simulink model "J2_PMSM_SimscapeRef"  (R2026b)
settings: Solver=ode23t  StopTime=0.3  MaxStep=1e-5  RelTol=1e-6  AbsTol=1e-8
model workspace (MAT data in the model file):
  p.pp = 8
  p.Rs = 0.04675
  p.Ld = 6.15e-05
  p.Lq = 6.15e-05
  p.Kt = 0.0436218747098
  p.psi = 0.00363515622582
  p.Jm = 1.7e-05
  p.IN = 10.4269458616
  p.nmax_rpm = 6000
  p.Vdc = 24
  p.Vmax = 12.4707658145
  p.Imax = 20.9
  p.Kp = 0.386415896392
  p.Ki = 293.738913111
  p.Kaw = 760.162601626
  p.N = 100
  p.JWG = 7.9e-06
  p.s = -1
  p.Kg = 14000
  p.zeta_g = 0.05
  p.cg = 5.90423576765
  p.J_test = 7.49e-05
libraries: fl_lib x9, nesl_utility x9, sl_discontinuities x1, ee_lib x1
settings Model: Creator=rninh  LastModifiedBy=rninh
settings SimscapeCC: SimscapeLogType=all  SimscapeNominalValues="[{\"value\":\"1\",\"unit\":\"A\"},{\"value\":\"1\",\"unit\":\"bar\"},{\"value\":\"1\",\"unit\":\"cm^2\"},{\"value\":\"1\",\"unit\":\"cm^3/s\"},{\"value\":\"1\",\"unit\":\"kJ/kg\"},{\"value\":\"1\",\"unit\":\"kW\"},{\"value\":\"1\",\"unit\":\"l\"},{\"value\":\"1\",\"unit\":\"N\"},{\"value\":\"1\",\"unit\":\"N*m\"},{\"value\":\"1\",\"unit\":\"V\"},{\"value\":\"0.001\",\"unit\":\"Wb\"}]"  SimscapeUseEnergyAccounting=off

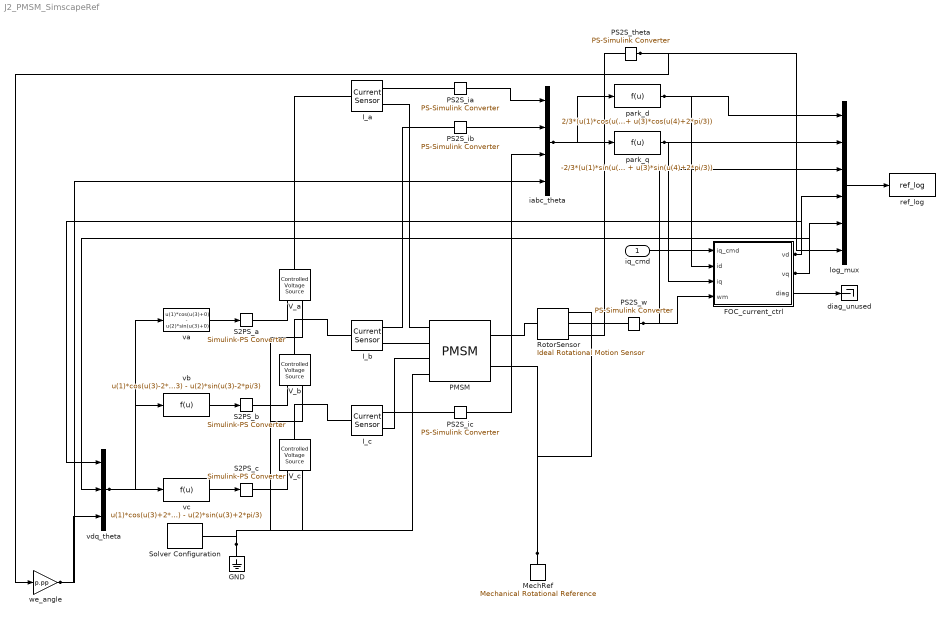
== system J2_PMSM_SimscapeRef ==
  iq_cmd : Inport  Interpolate=off
  FOC_current_ctrl : Subsystem
  GND : fl_lib/Electrical/Electrical Elements/Electrical Reference
  I_a : fl_lib/Electrical/Electrical Sensors/Current Sensor
  I_b : fl_lib/Electrical/Electrical Sensors/Current Sensor
  I_c : fl_lib/Electrical/Electrical Sensors/Current Sensor
  MechRef : fl_lib/Mechanical/Rotational Elements/Mechanical Rotational Reference
  PMSM : ee_lib/Electromechanical/Permanent Magnet/PMSM  port_option=ee.enum.threePhasePort.expanded  winding_type=ee.enum.electromech.statorconfiguration.wye  machine_param=ee.enum.pmsm.parameterization.constant  nPolePairs=p.pp  pmflux_param=ee.enum.pmflux.fluxlinkage  pm_flux_linkage=p.psi Wb  torque_constant=0.18 N*m/A  back_emf_constant=0.18 V*s/rad  stator_param=ee.enum.statorparam.LdLqL0  Ld=p.Ld H  Lq=p.Lq H  idVec=[-200, 0, 200] A  iqVec=[-200, 0, 200] A  LdMatrix=0.0002 * ones(3, 3) H  LqMatrix=0.0002 * ones(3, 3) H  PmMatrix=0.1 * ones(3, 3) Wb  ktMatrix=0.18 * ones(3, 3) N*m/A  keMatrix=0.18 * ones(3, 3) V*s/rad  L0=p.Ld H  Ls=0.0002 H  Lm=-0.00002 H  Ms=0.00002 H  Rs=p.Rs Ohm  zero_sequence=ee.enum.park.zerosequence.include  axes_param=ee.enum.rotorangle.daxis  loss_param=ee.enum.ironloss.none  losses_oc=[0, 0, 0] W  losses_sc=[0, 0, 0] W  f_losses=60 Hz  Isc_losses=95 A  J=p.J_test kg*m^2  lam=0 N*m*s/rad  i_d_specify=off  i_d_priority=None  i_d=0 A  i_d_nominal_specify=off  i_d_nominal_value=1  i_d_nominal_unit=A  i_q_specify=off  i_q_priority=None  i_q=0 A  i_q_nominal_specify=off  i_q_nominal_value=1  i_q_nominal_unit=A  torque_specify=off  torque_priority=None  torque=0 N*m  torque_nominal_specify=off  torque_nominal_value=1  torque_nominal_unit=N*m  angular_velocity_specify=off  angular_velocity_priority=High  angular_velocity=0 rpm  angular_velocity_nominal_specify=off  angular_velocity_nominal_value=1  angular_velocity_nominal_unit=rpm  angular_position_specify=off  angular_position_priority=High  angular_position=0 deg  angular_position_nominal_specify=off  angular_position_nominal_value=1  angular_position_nominal_unit=deg  alpha=3.93e-3 1/K  alpha_flux=-0.001 1/K  Tmeas=298.15 K  stator_thermal_mass=100 J/K  rotor_thermal_mass=200 J/K  Rm_percent_rotor=90  Rd_percent_rotor=30  temperatureA_specify=off  temperatureA_priority=High  temperatureA=25 degC  temperatureA_nominal_specify=off  temperatureA_nominal_value=1  temperatureA_nominal_unit=degC  temperatureB_specify=off  temperatureB_priority=High  temperatureB=25 degC  temperatureB_nominal_specify=off  temperatureB_nominal_value=1  temperatureB_nominal_unit=degC  temperatureC_specify=off  temperatureC_priority=High  temperatureC=25 degC  temperatureC_nominal_specify=off  temperatureC_nominal_value=1  temperatureC_nominal_unit=degC  temperatureR_specify=off  temperatureR_priority=High  temperatureR=25 degC  temperatureR_nominal_specify=off  temperatureR_nominal_value=1  temperatureR_nominal_unit=degC
  PS2S_ia : nesl_utility/PS-Simulink Converter  PhysicalDomain=network_engine_domain  SubClassName=ps_output  LeftPortType=input  RightPortType=output  PseudoPeriodic=off  Frequencies=[]  VectorFormat=inherit  Unit=A  AffineConversion=off
  PS2S_ib : nesl_utility/PS-Simulink Converter  PhysicalDomain=network_engine_domain  SubClassName=ps_output  LeftPortType=input  RightPortType=output  PseudoPeriodic=off  Frequencies=[]  VectorFormat=inherit  Unit=A  AffineConversion=off
  PS2S_ic : nesl_utility/PS-Simulink Converter  PhysicalDomain=network_engine_domain  SubClassName=ps_output  LeftPortType=input  RightPortType=output  PseudoPeriodic=off  Frequencies=[]  VectorFormat=inherit  Unit=A  AffineConversion=off
  PS2S_theta : nesl_utility/PS-Simulink Converter  PhysicalDomain=network_engine_domain  SubClassName=ps_output  LeftPortType=input  RightPortType=output  PseudoPeriodic=off  Frequencies=[]  VectorFormat=inherit  Unit=rad  AffineConversion=off
  PS2S_w : nesl_utility/PS-Simulink Converter  PhysicalDomain=network_engine_domain  SubClassName=ps_output  LeftPortType=input  RightPortType=output  PseudoPeriodic=off  Frequencies=[]  VectorFormat=inherit  Unit=rad/s  AffineConversion=off
  RotorSensor : fl_lib/Mechanical/Mechanical Sensors/Ideal Rotational Motion Sensor  reference=foundation.enum.MeasurementReference.difference  acceleration_port=false  velocity_port=true  position_port=true  wrap_angle=false  offset=0 rad
  S2PS_a : nesl_utility/Simulink-PS Converter  PhysicalDomain=network_engine_domain  SubClassName=ps_input  LeftPortType=input  RightPortType=output  PseudoPeriodic=off  Frequencies=[]  NoiseDistribution=none  NoiseParameters=[]  Unit=V  AffineConversion=off  FilteringAndDerivatives=zero  SimscapeFilterOrder=1  InputFilterTimeConstant=0.001  UdotUserProvided=0
  S2PS_b : nesl_utility/Simulink-PS Converter  PhysicalDomain=network_engine_domain  SubClassName=ps_input  LeftPortType=input  RightPortType=output  PseudoPeriodic=off  Frequencies=[]  NoiseDistribution=none  NoiseParameters=[]  Unit=V  AffineConversion=off  FilteringAndDerivatives=zero  SimscapeFilterOrder=1  InputFilterTimeConstant=0.001  UdotUserProvided=0
  S2PS_c : nesl_utility/Simulink-PS Converter  PhysicalDomain=network_engine_domain  SubClassName=ps_input  LeftPortType=input  RightPortType=output  PseudoPeriodic=off  Frequencies=[]  NoiseDistribution=none  NoiseParameters=[]  Unit=V  AffineConversion=off  FilteringAndDerivatives=zero  SimscapeFilterOrder=1  InputFilterTimeConstant=0.001  UdotUserProvided=0
  Solver Configuration : nesl_utility/Solver Configuration  PhysicalDomain=network_engine_domain  SubClassName=solver  LeftPortType=input  RightPortType=generic  Tones=[]  Harmonics=[]  SimulateNoise=off  Profile=off  UseLocalSampling=off  EnableSwitchedLinearOptims=on  FrequencyDomain=off  UseCCode=off  RelTol=0.001  AbsTol=0.001  MinStep=1e-09  ToWorkspace=off  RevertToSquareIcSolve=off  NumHomotopyIterations=100  PhasorMode=off  PhasorModeNumHarmonics=1  ConsistencySolver=NEWTON_XTOL_AFTER_FTOL  CanonicalOrdering=CANONICAL  OptimizeIntermediates=OPTIMIZED  MulticoreSolverChoice=BACKWARD_EULER  IndexReductionMethod=DerivativeReplacement  DoDC=off  ResidualTolerance=1e-09  ConsistencyTolSource=GLOBAL  ConsistencyAbsTol=0.001  ConsistencyRelTol=0.001  ConsistencyTolFactor=0.001  UseLocalSolver=off  LocalSolverChoice=NE_BACKWARD_EULER_ADVANCER  ResolveIndetEquations=on  FunctionEvalNumThread=1  LocalSolverSampleTime=0.001  DoFixedCost=off  MaxNonlinIter=3  MaxModeIter=2  ComputeImpulses=off  ImpulseIterations=2  LinearAlgebra=auto  LinearAlgebraNumThread=0  EquationFormulation=NE_TIME_EF  DelaysMemoryBudget=1024  AutomaticFiltering=on  FilteringTimeConstant=0.001  PartitionStorageMethod=AS_NEEDED  PartitionMemoryBudget=1024  PartitionMethod=BALANCED  MultibodyUseLocalSolver=off  MultibodyLocalSolverChoice=ODE1  MultibodyLocalSolverSampleTime=0.001
  V_a : fl_lib/Electrical/Electrical Sources/Controlled Voltage Source
  V_b : fl_lib/Electrical/Electrical Sources/Controlled Voltage Source
  V_c : fl_lib/Electrical/Electrical Sources/Controlled Voltage Source
  diag_unused : Terminator
  iabc_theta : Mux
  log_mux : Mux  Inputs=6
  park_d : Fcn  Expr=2/3*(u(1)*cos(u(4)) + u(2)*cos(u(4)-2*pi/3) + u(3)*cos(u(4)+2*pi/3))
  park_q : Fcn  Expr=-2/3*(u(1)*sin(u(4)) + u(2)*sin(u(4)-2*pi/3) + u(3)*sin(u(4)+2*pi/3))
  ref_log : ToWorkspace  VariableName=ref_log  SaveFormat=Timeseries  SampleTime=-1
  va : Fcn  Expr=u(1)*cos(u(3)+0) - u(2)*sin(u(3)+0)
  vb : Fcn  Expr=u(1)*cos(u(3)-2*pi/3) - u(2)*sin(u(3)-2*pi/3)
  vc : Fcn  Expr=u(1)*cos(u(3)+2*pi/3) - u(2)*sin(u(3)+2*pi/3)
  vdq_theta : Mux  Inputs=3
  we_angle : Gain  Gain=p.pp
  wires:
  vdq_theta/1 -> vb/1, vc/1, va/1
  we_angle/1 -> vdq_theta/3, iabc_theta/4
  log_mux/1 -> ref_log/1
  vc/1 -> S2PS_c/1
  va/1 -> S2PS_a/1
  vb/1 -> S2PS_b/1
  PS2S_w/1 -> log_mux/3, FOC_current_ctrl/4(wm)
  iabc_theta/1 -> park_d/1, park_q/1
  PS2S_ia/1 -> iabc_theta/1
  park_d/1 -> FOC_current_ctrl/2(id), log_mux/1
  PS2S_ib/1 -> iabc_theta/2
  PS2S_theta/1 -> we_angle/1, log_mux/6
  PS2S_ic/1 -> iabc_theta/3
  park_q/1 -> FOC_current_ctrl/3(iq), log_mux/2
  iq_cmd/1 -> FOC_current_ctrl/1(iq_cmd)
  FOC_current_ctrl/1(vd) -> vdq_theta/1, log_mux/4
  FOC_current_ctrl/2(vq) -> vdq_theta/2, log_mux/5
  FOC_current_ctrl/3(diag) -> diag_unused/1
  connections:
  S2PS_b/RConn1 -- V_b/RConn1
  S2PS_a/RConn1 -- V_a/RConn1
  S2PS_c/RConn1 -- V_c/RConn1
  GND/LConn1 -- V_a/RConn2 -- V_c/RConn2 -- V_b/RConn2 -- PMSM/LConn4 -- Solver Configuration/RConn1
  V_a/LConn1 -- I_a/LConn1
  V_b/LConn1 -- I_b/LConn1
  V_c/LConn1 -- I_c/LConn1
  I_a/RConn1 -- PS2S_ia/LConn1
  I_a/RConn2 -- PMSM/LConn1
  I_b/RConn1 -- PS2S_ib/LConn1
  I_b/RConn2 -- PMSM/LConn2
  I_c/RConn1 -- PS2S_ic/LConn1
  I_c/RConn2 -- PMSM/LConn3
  PMSM/RConn1 -- RotorSensor/LConn1
  PMSM/RConn2 -- MechRef/LConn1 -- RotorSensor/RConn1
  RotorSensor/RConn3 -- PS2S_theta/LConn1
  RotorSensor/RConn2 -- PS2S_w/LConn1

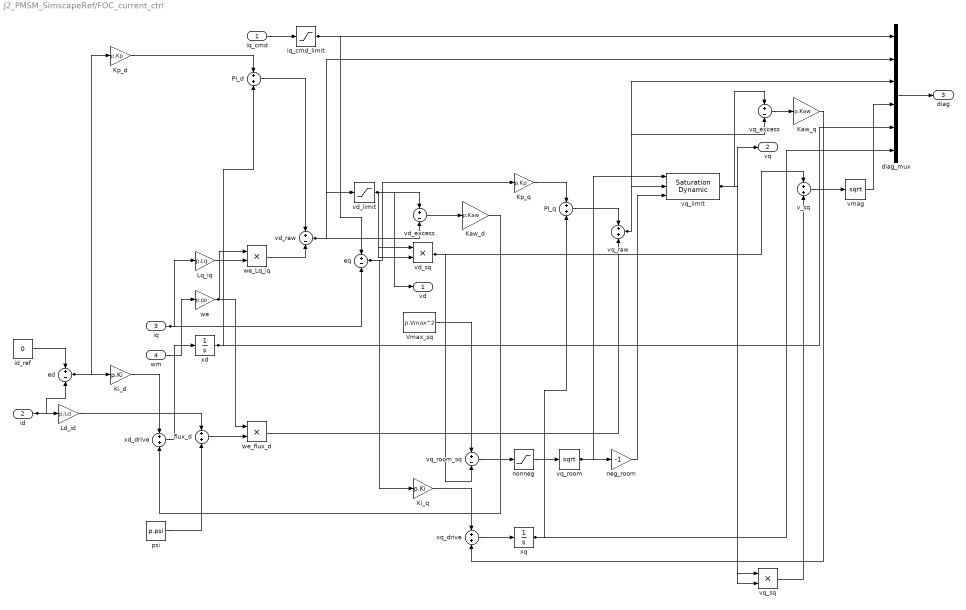
== system J2_PMSM_SimscapeRef/FOC_current_ctrl ==
  iq_cmd : Inport
  id : Inport  Port=2
  iq : Inport  Port=3
  wm : Inport  Port=4
  Kaw_d : Gain  Gain=p.Kaw
  Kaw_q : Gain  Gain=p.Kaw
  Ki_d : Gain  Gain=p.Ki
  Ki_q : Gain  Gain=p.Ki
  Kp_d : Gain  Gain=p.Kp
  Kp_q : Gain  Gain=p.Kp
  Ld_id : Gain  Gain=p.Ld
  Lq_iq : Gain  Gain=p.Lq
  PI_d : Sum
  PI_q : Sum
  Vmax_sq : Constant  Value=p.Vmax^2
  diag_mux : Mux  Inputs=6
  ed : Sum  Inputs=+-
  eq : Sum  Inputs=+-
  flux_d : Sum
  id_ref : Constant  Value=0
  iq_cmd_limit : Saturate  UpperLimit=p.Imax  LowerLimit=-p.Imax
  neg_room : Gain  Gain=-1
  nonneg : Saturate  UpperLimit=inf  LowerLimit=0
  psi : Constant  Value=p.psi
  v_sq : Sum
  vd_excess : Sum  Inputs=+-
  vd_limit : Saturate  UpperLimit=p.Vmax  LowerLimit=-p.Vmax
  vd_raw : Sum  Inputs=+-
  vd_sq : Product
  vmag : Sqrt
  vq_excess : Sum  Inputs=+-
  vq_limit : sl_discontinuities/Saturation Dynamic  OutMin=[]  OutMax=[]  OutDataTypeStr=Inherit: Same as second input  OutDataType=fixdt(1, 16)  OutScaling=2^-10  DoSatur=off
      settings: LibrarySourceBlock=|
      | simulink/Discontinuities/Saturation
      | Dynamic
  vq_raw : Sum
  vq_room : Sqrt
  vq_room_sq : Sum  Inputs=+-
  vq_sq : Product
  we : Gain  Gain=p.pp
  we_Lq_iq : Product
  we_flux_d : Product
  xd : Integrator
  xd_drive : Sum
  xq : Integrator
  xq_drive : Sum
  vd : Outport
  vq : Outport  Port=2
  diag : Outport  Port=3
  wires:
  vq_excess/1 -> Kaw_q/1
  vq_room/1 -> neg_room/1, vq_limit/1
  PI_q/1 -> vq_raw/1
  nonneg/1 -> vq_room/1
  vq_raw/1 -> vq_limit/2, diag_mux/3, vq_excess/2
  Kp_q/1 -> PI_q/1
  xq_drive/1 -> xq/1
  vq_room_sq/1 -> nonneg/1
  Kaw_d/1 -> xd_drive/2
  Ki_q/1 -> xq_drive/1
  Vmax_sq/1 -> vq_room_sq/1
  neg_room/1 -> vq_limit/3
  vd_sq/1 -> v_sq/1, vq_room_sq/2
  eq/1 -> Ki_q/1, Kp_q/1
  vq_limit/1 -> vq_sq/2, vq/1, vq_sq/1, vq_excess/1
  vd_limit/1 -> vd/1, vd_sq/1, vd_sq/2, vd_excess/1
  vd_raw/1 -> vd_limit/1, diag_mux/2, vd_excess/2
  we_Lq_iq/1 -> vd_raw/2
  vq_sq/1 -> v_sq/2
  PI_d/1 -> vd_raw/1
  xq/1 -> diag_mux/6, PI_q/2
  iq_cmd/1 -> iq_cmd_limit/1
  flux_d/1 -> we_flux_d/2
  Kaw_q/1 -> xq_drive/2
  xd/1 -> diag_mux/5, PI_d/2
  vd_excess/1 -> Kaw_d/1
  Lq_iq/1 -> we_Lq_iq/2
  v_sq/1 -> vmag/1
  psi/1 -> flux_d/2
  we_flux_d/1 -> vq_raw/2
  vmag/1 -> diag_mux/4
  diag_mux/1 -> diag/1
  xd_drive/1 -> xd/1
  iq/1 -> eq/2, Lq_iq/1
  Ki_d/1 -> xd_drive/1
  Ld_id/1 -> flux_d/1
  ed/1 -> Ki_d/1, Kp_d/1
  we/1 -> we_flux_d/1, we_Lq_iq/1
  Kp_d/1 -> PI_d/1
  id/1 -> Ld_id/1, ed/2
  id_ref/1 -> ed/1
  iq_cmd_limit/1 -> diag_mux/1, eq/1
  wm/1 -> we/1
